simulink model "space_vector_current_control"  (Simulink 7.5)
settings: Solver=ode23tb  StartTime=0.0  StopTime=0.2  FixedStep=1e-5  MaxStep=1e-4  RelTol=1e-4  AbsTol=1e-6
libraries: simulink x40, powerlib x35
settings Model: Creator=ankush  LastModifiedBy=ankush

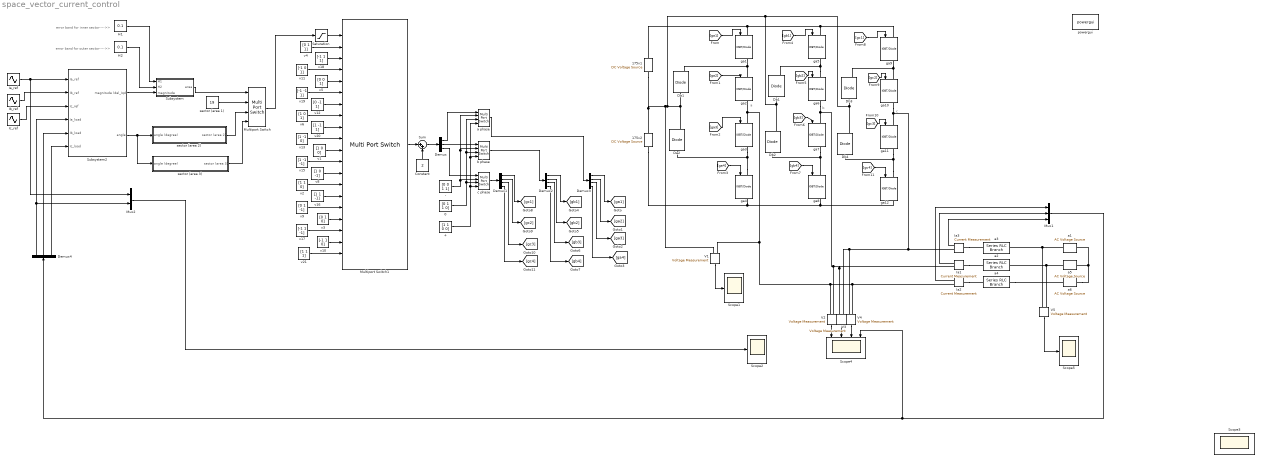
== system space_vector_current_control ==
  note: a
  note: b
  note: c
  note: error band for inner sector---->>
  note: error band for outer sector---->>
  + : Constant  Value=[1 1 0 0]  VectorParams1D=off  OutDataType=fixdt(1, 16)  OutScaling=2^0
  - : Constant  Value=[0 0 1 1]  OutDataType=fixdt(1, 16)  OutScaling=2^0
  0 : Constant  Value=[0 1 1 0]  OutDataType=fixdt(1, 16)  OutScaling=2^0
  175v1 : powerlib/Electrical Sources/DC Voltage Source  DialogController=POWERSYS.PowerSysDialog  SystemSampleTime=-1  Amplitude=300  Measurements=None
  175v2 : powerlib/Electrical Sources/DC Voltage Source  DialogController=POWERSYS.PowerSysDialog  SystemSampleTime=-1  Amplitude=300  Measurements=None
  Constant : Constant  Value=2  OutDataType=fixdt(1, 16)  OutScaling=2^0
  Da1 : powerlib/Power Electronics/Diode  DialogController=POWERSYS.PowerSysDialog  SystemSampleTime=-1  Ron=0.001  Lon=0  Vf=0.8  IC=0  UseSnubber=off  Rs=500  Cs=250e-9  Measurements=on
  Da2 : powerlib/Power Electronics/Diode  DialogController=POWERSYS.PowerSysDialog  SystemSampleTime=-1  Ron=0.001  Lon=0  Vf=0.8  IC=0  UseSnubber=off  Rs=500  Cs=250e-9  Measurements=on
  Db{1..4} (4 alike) : powerlib/Power Electronics/Diode  DialogController=POWERSYS.PowerSysDialog  SystemSampleTime=-1  Ron=0.001  Lon=0  Vf=0.8  IC=0  UseSnubber=off  Rs=500  Cs=250e-9  Measurements=on
  Demux : Demux  Outputs=3
  Demux1 : Demux
  Demux2 : Demux
  Demux3 : Demux
  Demux4 : Demux  Outputs=3
  H1 : Constant  Value=0.1  OutDataType=fixdt(1, 16)  OutScaling=2^0
  H2 : Constant  Value=0.1  OutDataType=fixdt(1, 16)  OutScaling=2^0
  Ia1 : powerlib/Measurements/Current Measurement  DialogController=POWERSYS.PowerSysDialog  SystemSampleTime=-1  PhasorSimulation=off  OutputType=Complex  PSBequivalent=0
  Ia2 : powerlib/Measurements/Current Measurement  DialogController=POWERSYS.PowerSysDialog  SystemSampleTime=-1  PhasorSimulation=off  OutputType=Complex  PSBequivalent=0
  Ia3 : powerlib/Measurements/Current Measurement  DialogController=POWERSYS.PowerSysDialog  SystemSampleTime=-1  PhasorSimulation=off  OutputType=Complex  PSBequivalent=0
  Ia_ref : Sin  Amplitude=5  Bias=0  Frequency=2*pi*50  Phase=0  Samples=10  SampleTime=0  Offset=0
  Ib_ref : Sin  Amplitude=5  Bias=0  Frequency=2*pi*50  Phase=-2*pi/3  Samples=10  SampleTime=0  Offset=0
  Ic_ref : Sin  Amplitude=5  Bias=0  Frequency=2*pi*50  Phase=2*pi/3  Samples=10  SampleTime=0  Offset=0
  Multiport Switch : MultiPortSwitch  zeroidx=off  OutDataType=fixdt(1, 16)  OutScaling=2^0
  Multiport Switch1 : MultiPortSwitch  Inputs=19  zeroidx=off  OutDataType=fixdt(1, 16)  OutScaling=2^0
  Mux1 : Mux  Inputs=3
  Mux2 : Mux  Inputs=2
  Saturation : Saturate  UpperLimit=19  LowerLimit=1  OutDataType=fixdt(1, 16)  OutScaling=2^0
  Scope1 : Scope
      settings: TimeRange=0.1  YMin=-200  YMax=175  SaveName=ScopeData3
  Scope2 : Scope
      settings: TimeRange=0.5  YMin=-5.5  YMax=5.5  SaveName=ScopeData2
  Scope3 : Scope  NumInputPorts=4
      settings: YMin=-5~-400~-350~-400  YMax=5~400~350~400
  Scope4 : Scope  NumInputPorts=4
      settings: YMin=-700~-700~-700~-7.5  YMax=700~700~700~7.5
  Scope5 : Scope
      settings: TimeRange=0.1  YMin=-600  YMax=600  SaveName=ScopeData6
  Subsystem : Subsystem
  Subsystem2 : Subsystem
  Sum : Sum  Inputs=|++  OutDataType=fixdt(1, 16)  OutScaling=2^0
  V{1..5} (5 alike) : powerlib/Measurements/Voltage Measurement  DialogController=POWERSYS.PowerSysDialog  SystemSampleTime=-1  PhasorSimulation=off  OutputType=Complex  PSBequivalent=0
  a phase : MultiPortSwitch  zeroidx=off  OutDataType=fixdt(1, 16)  OutScaling=2^0
  a1 : powerlib/Electrical Sources/AC Voltage Source  DialogController=POWERSYS.PowerSysDialog  SystemSampleTime=-1  Amplitude=240*sqrt(2)  Phase=120 + 88.178  Frequency=50  SampleTime=0  Measurements=None
  a2 : powerlib/Elements/Series RLC Branch  DialogController=POWERSYS.PowerSysDialog  PhysicalDomain=powersysdomain  SubClassName=unknown  LeftPortType=p1  RightPortType=p1  LConnTagsString=__new0  RConnTagsString=__new0  BranchType=RL  Resistance=0.03  Inductance=3e-3  SetiL0=off  InitialCurrent=0  Capacitance=2000e-6  Setx0=off  InitialVoltage=0  Measurements=None
  a3 : powerlib/Elements/Series RLC Branch  DialogController=POWERSYS.PowerSysDialog  PhysicalDomain=powersysdomain  SubClassName=unknown  LeftPortType=p1  RightPortType=p1  LConnTagsString=__new0  RConnTagsString=__new0  BranchType=RL  Resistance=0.03  Inductance=3e-3  SetiL0=off  InitialCurrent=0  Capacitance=2000e-6  Setx0=off  InitialVoltage=0  Measurements=None
  a4 : powerlib/Elements/Series RLC Branch  DialogController=POWERSYS.PowerSysDialog  PhysicalDomain=powersysdomain  SubClassName=unknown  LeftPortType=p1  RightPortType=p1  LConnTagsString=__new0  RConnTagsString=__new0  BranchType=RL  Resistance=0.03  Inductance=3e-3  SetiL0=off  InitialCurrent=0  Capacitance=2000e-6  Setx0=off  InitialVoltage=0  Measurements=None
  a5 : powerlib/Electrical Sources/AC Voltage Source  DialogController=POWERSYS.PowerSysDialog  SystemSampleTime=-1  Amplitude=240*sqrt(2)  Phase=-120 + 88.178  Frequency=50  SampleTime=0  Measurements=None
  a6 : powerlib/Electrical Sources/AC Voltage Source  DialogController=POWERSYS.PowerSysDialog  SystemSampleTime=-1  Amplitude=240*sqrt(2)  Phase=88.178  Frequency=50  SampleTime=0  Measurements=None
  b phase : MultiPortSwitch  zeroidx=off  OutDataType=fixdt(1, 16)  OutScaling=2^0
  c phase : MultiPortSwitch  zeroidx=off  OutDataType=fixdt(1, 16)  OutScaling=2^0
  ga{1..12} (12 alike) : powerlib/Power Electronics/IGBT//Diode  DialogController=POWERSYS.PowerSysDialog  SystemSampleTime=-1  Ron=1e-3  Rs=1e5  Cs=inf  Measurements=on
  powergui : powerlib/powergui  Priority=1  SystemSampleTime=-1  SimulationMode=Discrete  SampleTime=5e-6  frequency=60  SPID=off  DisableSnubberDevices=off  DisableRonSwitches=off  DisableVfSwitches=off  SwTol=0  Interpol=off  frequencyindice=0  echomessages=off  HookPort=off  DisplayEquations=off  FunctionMessages=off  EnableUseOfTLC=off  x0status=blocks  RestoreLinks=warning  ResistiveCurrentMeasurement=off  Ylog=off  Xlog=on  ShowGrid=off  save=off  variable=ZData  ZoomFFT=off  StartTime=0.0  cycles=1  DisplayStyle=1  FreqAxis=off  MaxFrequency=1000  frequencyindicesteady=1  display=off  methode=off
  sector (area 1) : Constant  Value=19  OutDataType=fixdt(1, 16)  OutScaling=2^0
  sector (area 2) : Subsystem
  sector (area 3) : Subsystem
  v1 : Constant  Value=[1 0 0]  VectorParams1D=off  OutDataType=fixdt(1, 16)  OutScaling=2^0
  v10 : Constant  Value=[-1 1 0]  VectorParams1D=off  OutDataType=fixdt(1, 16)  OutScaling=2^0
  v11 : Constant  Value=[-1 0 1]  VectorParams1D=off  OutDataType=fixdt(1, 16)  OutScaling=2^0
  v12 : Constant  Value=[0 -1 1]  VectorParams1D=off  OutDataType=fixdt(1, 16)  OutScaling=2^0
  v13 : Constant  Value=[1 -1 0]  VectorParams1D=off  OutDataType=fixdt(1, 16)  OutScaling=2^0
  v15 : Constant  Value=[1 -1 -1]  VectorParams1D=off  OutDataType=fixdt(1, 16)  OutScaling=2^0
  v16 : Constant  Value=[1 1 -1]  VectorParams1D=off  OutDataType=fixdt(1, 16)  OutScaling=2^0
  v17 : Constant  Value=[-1 1 -1]  VectorParams1D=off  OutDataType=fixdt(1, 16)  OutScaling=2^0
  v18 : Constant  Value=[-1 1 1]  VectorParams1D=off  OutDataType=fixdt(1, 16)  OutScaling=2^0
  v19 : Constant  Value=[-1 -1 1]  VectorParams1D=off  OutDataType=fixdt(1, 16)  OutScaling=2^0
  v2 : Constant  Value=[1 1 0]  VectorParams1D=off  OutDataType=fixdt(1, 16)  OutScaling=2^0
  v20 : Constant  Value=[1 -1 1]  VectorParams1D=off  OutDataType=fixdt(1, 16)  OutScaling=2^0
  v21 : Constant  Value=[1 1 1]  VectorParams1D=off  OutDataType=fixdt(1, 16)  OutScaling=2^0
  v3 : Constant  Value=[0 1 0]  VectorParams1D=off  OutDataType=fixdt(1, 16)  OutScaling=2^0
  v4 : Constant  Value=[0 1 1]  VectorParams1D=off  OutDataType=fixdt(1, 16)  OutScaling=2^0
  v5 : Constant  Value=[0 0 1]  VectorParams1D=off  OutDataType=fixdt(1, 16)  OutScaling=2^0
  v6 : Constant  Value=[1 0 1]  VectorParams1D=off  OutDataType=fixdt(1, 16)  OutScaling=2^0
  v8 : Constant  Value=[1 0 -1]  VectorParams1D=off  OutDataType=fixdt(1, 16)  OutScaling=2^0
  v9 : Constant  Value=[0 1 -1]  VectorParams1D=off  OutDataType=fixdt(1, 16)  OutScaling=2^0
  wires:
  sector (area 1)/1 -> Multiport Switch/2
  sector (area 2)/1(sector (area 2)) -> Multiport Switch/3
  sector (area 3)/1(sector (area 3)) -> Multiport Switch/4
  Multiport Switch/1 -> Saturation/1
  Ia_ref/1 -> Mux2/1, Subsystem2/1(Ia_ref)
  Ib_ref/1 -> Subsystem2/2(Ib_ref)
  Ic_ref/1 -> Subsystem2/3(Ic_ref)
  Sum/1 -> Demux/1
  Demux/2 -> b phase/1
  +/1 -> c phase/4, b phase/4, a phase/4
  0/1 -> c phase/3, a phase/3, b phase/3
  -/1 -> a phase/2, b phase/2, c phase/2
  c phase/1 -> Demux1/1
  Demux1/1 -> [gc1]
  Demux1/4 -> [gc4]
  b phase/1 -> Demux2/1
  Demux1/2 -> [gc2]
  Demux1/3 -> [gc3]
  Demux2/4 -> [gb4]
  Demux2/3 -> [gb3]
  Demux2/2 -> [gb2]
  Demux2/1 -> [gb1]
  a phase/1 -> Demux3/1
  Demux3/4 -> [ga4]
  Demux3/3 -> [ga3]
  Demux3/2 -> [ga2]
  Demux3/1 -> [ga1]
  Constant/1 -> Sum/2
  Multiport Switch1/1 -> Sum/1
  [ga1] -> ga1/1
  [ga2] -> ga2/1
  [ga3] -> ga3/1
  [ga4] -> ga4/1
  [gb1] -> ga5/1
  [gb2] -> ga6/1
  [gb3] -> ga7/1
  [gb4] -> ga8/1
  [gc1] -> ga9/1
  [gc2] -> ga10/1
  [gc3] -> ga11/1
  [gc4] -> ga12/1
  V4/1 -> Scope4/3
  V3/1 -> Scope4/2
  V2/1 -> Scope4/1
  Subsystem2/1(magnitude (del_Iqd)) -> Subsystem/3(magnitude)
  v10/1 -> Multiport Switch1/19
  v17/1 -> Multiport Switch1/18
  v9/1 -> Multiport Switch1/16
  v16/1 -> Multiport Switch1/15
  v8/1 -> Multiport Switch1/13
  v15/1 -> Multiport Switch1/12
  v13/1 -> Multiport Switch1/10
  v20/1 -> Multiport Switch1/9
  v12/1 -> Multiport Switch1/7
  v19/1 -> Multiport Switch1/6
  v11/1 -> Multiport Switch1/4
  v18/1 -> Multiport Switch1/3
  v3/1 -> Multiport Switch1/17
  v2/1 -> Multiport Switch1/14
  v1/1 -> Multiport Switch1/11
  v6/1 -> Multiport Switch1/8
  v5/1 -> Multiport Switch1/5
  v4/1 -> Multiport Switch1/2
  Mux2/1 -> Scope2/1
  Demux/3 -> c phase/1
  Demux/1 -> a phase/1
  v21/1 -> Multiport Switch1/20
  Saturation/1 -> Multiport Switch1/1
  Demux4/1 -> Subsystem2/4(Ia_load), Mux2/2
  Demux4/2 -> Subsystem2/5(Ib_load)
  Demux4/3 -> Subsystem2/6(Ic_load)
  H1/1 -> Subsystem/1(H1)
  H2/1 -> Subsystem/2(H2)
  Subsystem2/2(angle) -> sector (area 2)/1(angle (degree)), sector (area 3)/1(angle (degree))
  Subsystem/1(area) -> Multiport Switch/1
  V1/1 -> Scope1/1
  Mux1/1 -> Demux4/1, Scope4/4
  Ia2/1 -> Mux1/1
  Ia1/1 -> Mux1/2
  Ia3/1 -> Mux1/3
  V5/1 -> Scope5/1
  connections:
  ga1/RConn1 -- Da1/RConn1 -- ga2/LConn1
  ga4/LConn1 -- Da2/LConn1 -- ga3/RConn1
  175v1/RConn1 -- ga1/LConn1 -- ga5/LConn1 -- ga9/LConn1
  ga12/RConn1 -- ga4/RConn1 -- 175v2/LConn1 -- ga8/RConn1
  ga6/LConn1 -- Db1/RConn1 -- ga5/RConn1
  Db2/LConn1 -- ga8/LConn1 -- ga7/RConn1
  Db3/RConn1 -- ga10/LConn1 -- ga9/RConn1
  ga12/LConn1 -- Db4/LConn1 -- ga11/RConn1
  V3/LConn2 -- V4/LConn1 -- ga10/RConn1 -- ga11/LConn1 -- Ia3/RConn1
  V4/LConn2 -- ga3/LConn1 -- ga2/RConn1 -- V1/LConn2 -- V2/LConn1 -- Ia2/RConn1
  V3/LConn1 -- ga7/LConn1 -- ga6/RConn1 -- V2/LConn2 -- Ia1/RConn1
  175v1/LConn1 -- 175v2/RConn1 -- Db3/LConn1 -- Db4/RConn1 -- Db2/RConn1 -- Db1/LConn1 -- Da2/RConn1 -- Da1/LConn1 -- V1/LConn1
  a6/LConn1 -- a1/LConn1 -- a5/LConn1
  Ia3/LConn1 -- a3/RConn1
  Ia2/LConn1 -- a4/RConn1
  Ia1/LConn1 -- a2/RConn1
  a4/LConn1 -- a6/RConn1
  a5/RConn1 -- a2/LConn1 -- V5/LConn2
  a1/RConn1 -- a3/LConn1 -- V5/LConn1

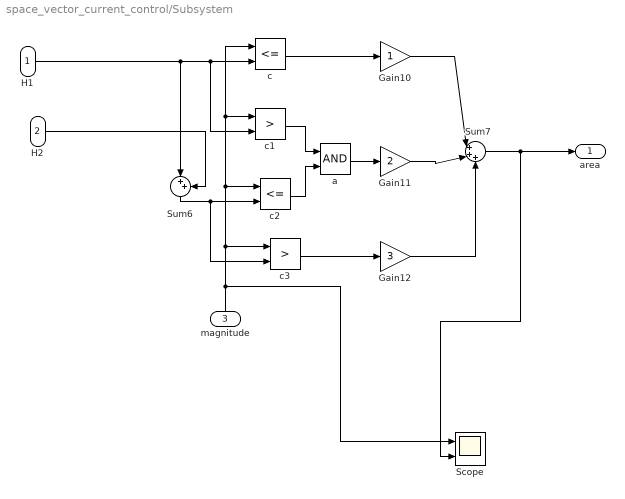
== system space_vector_current_control/Subsystem ==
  H1 : Inport
  H2 : Inport  Port=2
  magnitude : Inport  Port=3
  Gain10 : Gain  ParameterDataType=fixdt(1, 16)  ParameterScaling=2^0  OutDataType=fixdt(1, 16)  OutScaling=2^0
  Gain11 : Gain  Gain=2  ParameterDataType=fixdt(1, 16)  ParameterScaling=2^0  OutDataType=fixdt(1, 16)  OutScaling=2^0
  Gain12 : Gain  Gain=3  ParameterDataType=fixdt(1, 16)  ParameterScaling=2^0  OutDataType=fixdt(1, 16)  OutScaling=2^0
  Scope : Scope  NumInputPorts=2
      settings: YMin=-1.73472e-017~1  YMax=0.23~3  SaveName=ScopeData4
  Sum6 : Sum  Inputs=|++  OutDataType=fixdt(1, 16)  OutScaling=2^0
  Sum7 : Sum  Inputs=|+++  OutDataType=fixdt(1, 16)  OutScaling=2^0
  a : Logic  AllPortsSameDT=off  OutDataTypeMode=boolean  LogicDataType=fixdt(0, 8)  OutDataTypeStr=boolean
  c : RelationalOperator  Operator=<=  LogicOutDataTypeMode=boolean  LogicDataType=fixdt(0, 8)  OutDataTypeStr=boolean
  c1 : RelationalOperator  Operator=>  LogicOutDataTypeMode=boolean  LogicDataType=fixdt(0, 8)  OutDataTypeStr=boolean
  c2 : RelationalOperator  Operator=<=  LogicOutDataTypeMode=boolean  LogicDataType=fixdt(0, 8)  OutDataTypeStr=boolean
  c3 : RelationalOperator  Operator=>  LogicOutDataTypeMode=boolean  LogicDataType=fixdt(0, 8)  OutDataTypeStr=boolean
  area : Outport
  wires:
  H1/1 -> Sum6/1, c/2, c1/2
  c/1 -> Gain10/1
  H2/1 -> Sum6/2
  Sum6/1 -> c2/2, c3/2
  c1/1 -> a/1
  c2/1 -> a/2
  a/1 -> Gain11/1
  c3/1 -> Gain12/1
  Gain10/1 -> Sum7/1
  Gain11/1 -> Sum7/2
  Gain12/1 -> Sum7/3
  magnitude/1 -> c/1, c1/1, c2/1, c3/1, Scope/1
  Sum7/1 -> area/1, Scope/2

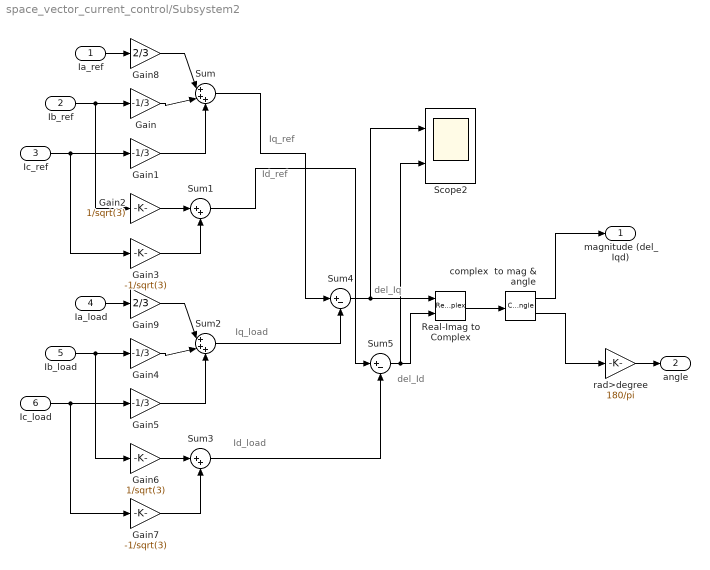
== system space_vector_current_control/Subsystem2 ==
  note: Iq_ref
  note: Id_ref
  note: Iq_load
  note: Id_load
  note: del_Iq
  note: del_Id
  Ia_ref : Inport
  Ib_ref : Inport  Port=2
  Ic_ref : Inport  Port=3
  Ia_load : Inport  Port=4
  Ib_load : Inport  Port=5
  Ic_load : Inport  Port=6
  Gain{,1,4..5} (4 alike) : Gain  Gain=-1/3  ParameterDataType=fixdt(1, 16)  ParameterScaling=2^0  OutDataType=fixdt(1, 16)  OutScaling=2^0
  Gain2 : Gain  Gain=1/sqrt(3)  ParameterDataType=fixdt(1, 16)  ParameterScaling=2^0  OutDataType=fixdt(1, 16)  OutScaling=2^0
  Gain3 : Gain  Gain=-1/sqrt(3)  ParameterDataType=fixdt(1, 16)  ParameterScaling=2^0  OutDataType=fixdt(1, 16)  OutScaling=2^0
  Gain6 : Gain  Gain=1/sqrt(3)  ParameterDataType=fixdt(1, 16)  ParameterScaling=2^0  OutDataType=fixdt(1, 16)  OutScaling=2^0
  Gain7 : Gain  Gain=-1/sqrt(3)  ParameterDataType=fixdt(1, 16)  ParameterScaling=2^0  OutDataType=fixdt(1, 16)  OutScaling=2^0
  Gain8 : Gain  Gain=2/3  ParameterDataType=fixdt(1, 16)  ParameterScaling=2^0  OutDataType=fixdt(1, 16)  OutScaling=2^0
  Gain9 : Gain  Gain=2/3  ParameterDataType=fixdt(1, 16)  ParameterScaling=2^0  OutDataType=fixdt(1, 16)  OutScaling=2^0
  Real-Imag to Complex : RealImagToComplex
  Scope2 : Scope  NumInputPorts=2
      settings: YMin=0.5~-12  YMax=9~-1.5  SaveName=ScopeData5
  Sum : Sum  Inputs=|+++  OutDataType=fixdt(1, 16)  OutScaling=2^0
  Sum1 : Sum  Inputs=|++  OutDataType=fixdt(1, 16)  OutScaling=2^0
  Sum2 : Sum  Inputs=|+++  OutDataType=fixdt(1, 16)  OutScaling=2^0
  Sum3 : Sum  Inputs=|++  OutDataType=fixdt(1, 16)  OutScaling=2^0
  Sum4 : Sum  Inputs=|+-  OutDataType=fixdt(1, 16)  OutScaling=2^0
  Sum5 : Sum  Inputs=|+-  OutDataType=fixdt(1, 16)  OutScaling=2^0
  complex  to mag & angle : ComplexToMagnitudeAngle
  rad>degree : Gain  Gain=180/pi  ParameterDataType=fixdt(1, 16)  ParameterScaling=2^0  OutDataType=fixdt(1, 16)  OutScaling=2^0
  magnitude (del_Iqd) : Outport
  angle : Outport  Port=2
  wires:
  Gain/1 -> Sum/2
  Gain1/1 -> Sum/3
  Ib_ref/1 -> Gain2/1, Gain/1
  Ic_ref/1 -> Gain3/1, Gain1/1
  Gain2/1 -> Sum1/1
  Gain3/1 -> Sum1/2
  Sum/1 -> Sum4/1
  Sum1/1 -> Sum5/1
  Gain4/1 -> Sum2/2
  Gain5/1 -> Sum2/3
  Ib_load/1 -> Gain4/1, Gain6/1
  Ic_load/1 -> Gain5/1, Gain7/1
  Gain6/1 -> Sum3/1
  Gain7/1 -> Sum3/2
  Sum2/1 -> Sum4/2
  Sum3/1 -> Sum5/2
  Real-Imag to Complex/1 -> complex  to mag & angle/1
  Sum4/1 -> Real-Imag to Complex/1, Scope2/1
  Sum5/1 -> Real-Imag to Complex/2, Scope2/2
  Gain8/1 -> Sum/1
  Gain9/1 -> Sum2/1
  Ia_ref/1 -> Gain8/1
  Ia_load/1 -> Gain9/1
  rad>degree/1 -> angle/1
  complex  to mag & angle/2 -> rad>degree/1
  complex  to mag & angle/1 -> magnitude (del_Iqd)/1

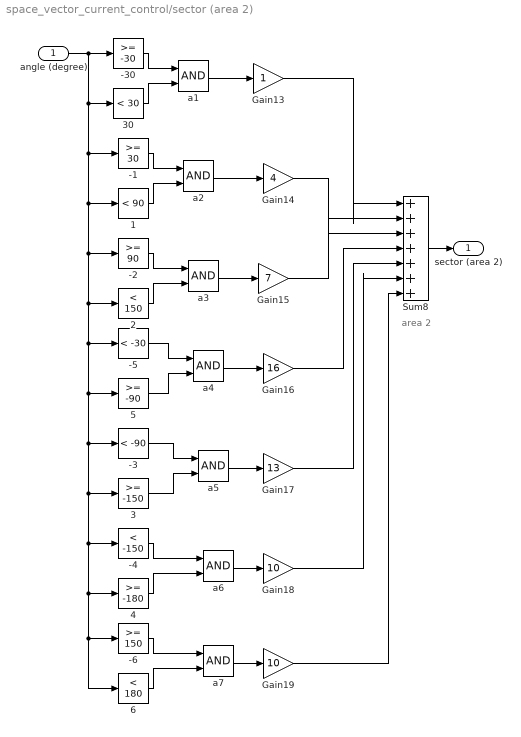
== system space_vector_current_control/sector (area 2) ==
  note: area 2
  angle (degree) : Inport
  -1 : simulink/Logic and Bit Operations/Compare To Constant  SystemSampleTime=-1  relop=>=  const=30  LogicOutDataTypeMode=uint8
  -2 : simulink/Logic and Bit Operations/Compare To Constant  SystemSampleTime=-1  relop=>=  const=90  LogicOutDataTypeMode=uint8
  -3 : simulink/Logic and Bit Operations/Compare To Constant  SystemSampleTime=-1  relop=<  const=-90  LogicOutDataTypeMode=uint8
  -30 : simulink/Logic and Bit Operations/Compare To Constant  SystemSampleTime=-1  relop=>=  const=-30  LogicOutDataTypeMode=uint8
  -4 : simulink/Logic and Bit Operations/Compare To Constant  SystemSampleTime=-1  relop=<  const=-150  LogicOutDataTypeMode=uint8
  -5 : simulink/Logic and Bit Operations/Compare To Constant  SystemSampleTime=-1  relop=<  const=-30  LogicOutDataTypeMode=uint8
  -6 : simulink/Logic and Bit Operations/Compare To Constant  SystemSampleTime=-1  relop=>=  const=150  LogicOutDataTypeMode=uint8
  1 : simulink/Logic and Bit Operations/Compare To Constant  SystemSampleTime=-1  relop=<  const=90  LogicOutDataTypeMode=uint8
  2 : simulink/Logic and Bit Operations/Compare To Constant  SystemSampleTime=-1  relop=<  const=150  LogicOutDataTypeMode=uint8
  3 : simulink/Logic and Bit Operations/Compare To Constant  SystemSampleTime=-1  relop=>=  const=-150  LogicOutDataTypeMode=uint8
  30 : simulink/Logic and Bit Operations/Compare To Constant  SystemSampleTime=-1  relop=<  const=30  LogicOutDataTypeMode=uint8
  4 : simulink/Logic and Bit Operations/Compare To Constant  SystemSampleTime=-1  relop=>=  const=-180  LogicOutDataTypeMode=uint8
  5 : simulink/Logic and Bit Operations/Compare To Constant  SystemSampleTime=-1  relop=>=  const=-90  LogicOutDataTypeMode=uint8
  6 : simulink/Logic and Bit Operations/Compare To Constant  SystemSampleTime=-1  relop=<  const=180  LogicOutDataTypeMode=uint8
  Gain13 : Gain  ParameterDataType=fixdt(1, 16)  ParameterScaling=2^0  OutDataType=fixdt(1, 16)  OutScaling=2^0
  Gain14 : Gain  Gain=4  ParameterDataType=fixdt(1, 16)  ParameterScaling=2^0  OutDataType=fixdt(1, 16)  OutScaling=2^0
  Gain15 : Gain  Gain=7  ParameterDataType=fixdt(1, 16)  ParameterScaling=2^0  OutDataType=fixdt(1, 16)  OutScaling=2^0
  Gain16 : Gain  Gain=16  ParameterDataType=fixdt(1, 16)  ParameterScaling=2^0  OutDataType=fixdt(1, 16)  OutScaling=2^0
  Gain17 : Gain  Gain=13  ParameterDataType=fixdt(1, 16)  ParameterScaling=2^0  OutDataType=fixdt(1, 16)  OutScaling=2^0
  Gain18 : Gain  Gain=10  ParameterDataType=fixdt(1, 16)  ParameterScaling=2^0  OutDataType=fixdt(1, 16)  OutScaling=2^0
  Gain19 : Gain  Gain=10  ParameterDataType=fixdt(1, 16)  ParameterScaling=2^0  OutDataType=fixdt(1, 16)  OutScaling=2^0
  Sum8 : Sum  Inputs=|+++++++  OutDataType=fixdt(1, 16)  OutScaling=2^0
  a{1..7} (7 alike) : Logic  AllPortsSameDT=off  OutDataTypeMode=boolean  LogicDataType=fixdt(0, 8)  OutDataTypeStr=boolean
  sector (area 2) : Outport
  wires:
  -30/1 -> a1/1
  30/1 -> a1/2
  -1/1 -> a2/1
  1/1 -> a2/2
  -2/1 -> a3/1
  2/1 -> a3/2
  -5/1 -> a4/1
  5/1 -> a4/2
  -3/1 -> a5/1
  3/1 -> a5/2
  -4/1 -> a6/1
  4/1 -> a6/2
  a1/1 -> Gain13/1
  a2/1 -> Gain14/1
  a3/1 -> Gain15/1
  a4/1 -> Gain16/1
  a5/1 -> Gain17/1
  a6/1 -> Gain18/1
  Gain13/1 -> Sum8/1
  Gain14/1 -> Sum8/2
  Gain15/1 -> Sum8/3
  Gain16/1 -> Sum8/4
  Gain17/1 -> Sum8/5
  Gain18/1 -> Sum8/6
  -6/1 -> a7/1
  6/1 -> a7/2
  a7/1 -> Gain19/1
  Gain19/1 -> Sum8/7
  angle (degree)/1 -> -30/1, 30/1, -1/1, 1/1, -2/1, 2/1, -5/1, 5/1, -3/1, 3/1, -4/1, 4/1, -6/1, 6/1
  Sum8/1 -> sector (area 2)/1

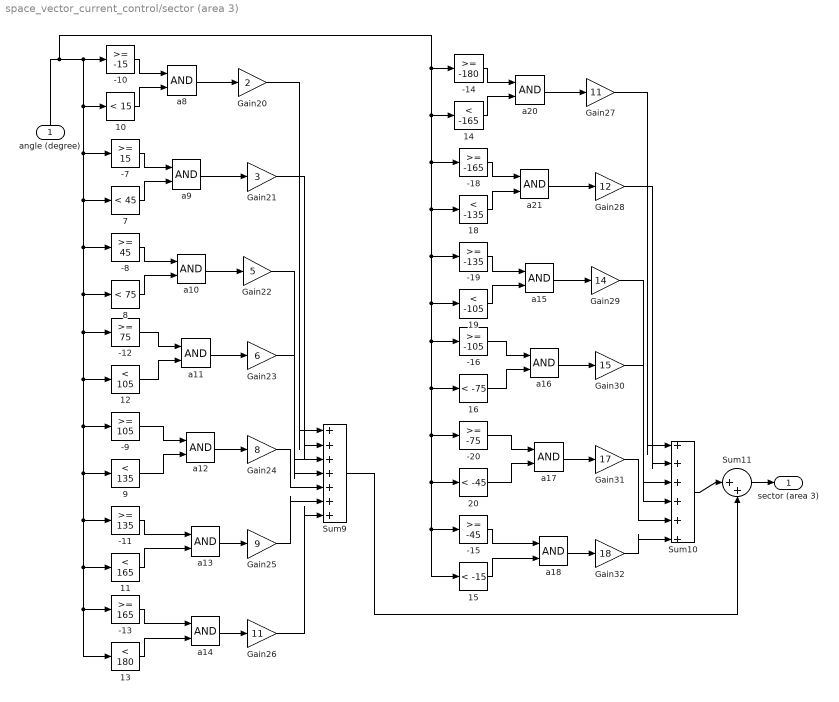
== system space_vector_current_control/sector (area 3) ==
  angle (degree) : Inport
  -10 : simulink/Logic and Bit Operations/Compare To Constant  SystemSampleTime=-1  relop=>=  const=-15  LogicOutDataTypeMode=uint8
  -11 : simulink/Logic and Bit Operations/Compare To Constant  SystemSampleTime=-1  relop=>=  const=135  LogicOutDataTypeMode=uint8
  -12 : simulink/Logic and Bit Operations/Compare To Constant  SystemSampleTime=-1  relop=>=  const=75  LogicOutDataTypeMode=uint8
  -13 : simulink/Logic and Bit Operations/Compare To Constant  SystemSampleTime=-1  relop=>=  const=165  LogicOutDataTypeMode=uint8
  -14 : simulink/Logic and Bit Operations/Compare To Constant  SystemSampleTime=-1  relop=>=  const=-180  LogicOutDataTypeMode=uint8
  -15 : simulink/Logic and Bit Operations/Compare To Constant  SystemSampleTime=-1  relop=>=  const=-45  LogicOutDataTypeMode=uint8
  -16 : simulink/Logic and Bit Operations/Compare To Constant  SystemSampleTime=-1  relop=>=  const=-105  LogicOutDataTypeMode=uint8
  -18 : simulink/Logic and Bit Operations/Compare To Constant  SystemSampleTime=-1  relop=>=  const=-165  LogicOutDataTypeMode=uint8
  -19 : simulink/Logic and Bit Operations/Compare To Constant  SystemSampleTime=-1  relop=>=  const=-135  LogicOutDataTypeMode=uint8
  -20 : simulink/Logic and Bit Operations/Compare To Constant  SystemSampleTime=-1  relop=>=  const=-75  LogicOutDataTypeMode=uint8
  -7 : simulink/Logic and Bit Operations/Compare To Constant  SystemSampleTime=-1  relop=>=  const=15  LogicOutDataTypeMode=uint8
  -8 : simulink/Logic and Bit Operations/Compare To Constant  SystemSampleTime=-1  relop=>=  const=45  LogicOutDataTypeMode=uint8
  -9 : simulink/Logic and Bit Operations/Compare To Constant  SystemSampleTime=-1  relop=>=  const=105  LogicOutDataTypeMode=uint8
  10 : simulink/Logic and Bit Operations/Compare To Constant  SystemSampleTime=-1  relop=<  const=15  LogicOutDataTypeMode=uint8
  11 : simulink/Logic and Bit Operations/Compare To Constant  SystemSampleTime=-1  relop=<  const=165  LogicOutDataTypeMode=uint8
  12 : simulink/Logic and Bit Operations/Compare To Constant  SystemSampleTime=-1  relop=<  const=105  LogicOutDataTypeMode=uint8
  13 : simulink/Logic and Bit Operations/Compare To Constant  SystemSampleTime=-1  relop=<  const=180  LogicOutDataTypeMode=uint8
  14 : simulink/Logic and Bit Operations/Compare To Constant  SystemSampleTime=-1  relop=<  const=-165  LogicOutDataTypeMode=uint8
  15 : simulink/Logic and Bit Operations/Compare To Constant  SystemSampleTime=-1  relop=<  const=-15  LogicOutDataTypeMode=uint8
  16 : simulink/Logic and Bit Operations/Compare To Constant  SystemSampleTime=-1  relop=<  const=-75  LogicOutDataTypeMode=uint8
  18 : simulink/Logic and Bit Operations/Compare To Constant  SystemSampleTime=-1  relop=<  const=-135  LogicOutDataTypeMode=uint8
  19 : simulink/Logic and Bit Operations/Compare To Constant  SystemSampleTime=-1  relop=<  const=-105  LogicOutDataTypeMode=uint8
  20 : simulink/Logic and Bit Operations/Compare To Constant  SystemSampleTime=-1  relop=<  const=-45  LogicOutDataTypeMode=uint8
  7 : simulink/Logic and Bit Operations/Compare To Constant  SystemSampleTime=-1  relop=<  const=45  LogicOutDataTypeMode=uint8
  8 : simulink/Logic and Bit Operations/Compare To Constant  SystemSampleTime=-1  relop=<  const=75  LogicOutDataTypeMode=uint8
  9 : simulink/Logic and Bit Operations/Compare To Constant  SystemSampleTime=-1  relop=<  const=135  LogicOutDataTypeMode=uint8
  Gain20 : Gain  Gain=2  ParameterDataType=fixdt(1, 16)  ParameterScaling=2^0  OutDataType=fixdt(1, 16)  OutScaling=2^0
  Gain21 : Gain  Gain=3  ParameterDataType=fixdt(1, 16)  ParameterScaling=2^0  OutDataType=fixdt(1, 16)  OutScaling=2^0
  Gain22 : Gain  Gain=5  ParameterDataType=fixdt(1, 16)  ParameterScaling=2^0  OutDataType=fixdt(1, 16)  OutScaling=2^0
  Gain23 : Gain  Gain=6  ParameterDataType=fixdt(1, 16)  ParameterScaling=2^0  OutDataType=fixdt(1, 16)  OutScaling=2^0
  Gain24 : Gain  Gain=8  ParameterDataType=fixdt(1, 16)  ParameterScaling=2^0  OutDataType=fixdt(1, 16)  OutScaling=2^0
  Gain25 : Gain  Gain=9  ParameterDataType=fixdt(1, 16)  ParameterScaling=2^0  OutDataType=fixdt(1, 16)  OutScaling=2^0
  Gain26 : Gain  Gain=11  ParameterDataType=fixdt(1, 16)  ParameterScaling=2^0  OutDataType=fixdt(1, 16)  OutScaling=2^0
  Gain27 : Gain  Gain=11  ParameterDataType=fixdt(1, 16)  ParameterScaling=2^0  OutDataType=fixdt(1, 16)  OutScaling=2^0
  Gain28 : Gain  Gain=12  ParameterDataType=fixdt(1, 16)  ParameterScaling=2^0  OutDataType=fixdt(1, 16)  OutScaling=2^0
  Gain29 : Gain  Gain=14  ParameterDataType=fixdt(1, 16)  ParameterScaling=2^0  OutDataType=fixdt(1, 16)  OutScaling=2^0
  Gain30 : Gain  Gain=15  ParameterDataType=fixdt(1, 16)  ParameterScaling=2^0  OutDataType=fixdt(1, 16)  OutScaling=2^0
  Gain31 : Gain  Gain=17  ParameterDataType=fixdt(1, 16)  ParameterScaling=2^0  OutDataType=fixdt(1, 16)  OutScaling=2^0
  Gain32 : Gain  Gain=18  ParameterDataType=fixdt(1, 16)  ParameterScaling=2^0  OutDataType=fixdt(1, 16)  OutScaling=2^0
  Sum10 : Sum  Inputs=|++++++  OutDataType=fixdt(1, 16)  OutScaling=2^0
  Sum11 : Sum  Inputs=|++  OutDataType=fixdt(1, 16)  OutScaling=2^0
  Sum9 : Sum  Inputs=|+++++++  OutDataType=fixdt(1, 16)  OutScaling=2^0
  a{8..18,20..21} (13 alike) : Logic  AllPortsSameDT=off  OutDataTypeMode=boolean  LogicDataType=fixdt(0, 8)  OutDataTypeStr=boolean
  sector (area 3) : Outport
  wires:
  -10/1 -> a8/1
  10/1 -> a8/2
  -7/1 -> a9/1
  7/1 -> a9/2
  -8/1 -> a10/1
  8/1 -> a10/2
  -12/1 -> a11/1
  12/1 -> a11/2
  -9/1 -> a12/1
  9/1 -> a12/2
  -11/1 -> a13/1
  11/1 -> a13/2
  a8/1 -> Gain20/1
  a9/1 -> Gain21/1
  a10/1 -> Gain22/1
  a11/1 -> Gain23/1
  a12/1 -> Gain24/1
  a13/1 -> Gain25/1
  -13/1 -> a14/1
  13/1 -> a14/2
  a14/1 -> Gain26/1
  Gain20/1 -> Sum9/1
  Gain21/1 -> Sum9/2
  Gain22/1 -> Sum9/3
  Gain23/1 -> Sum9/4
  Gain24/1 -> Sum9/5
  Gain25/1 -> Sum9/6
  Gain26/1 -> Sum9/7
  -14/1 -> a20/1
  14/1 -> a20/2
  -18/1 -> a21/1
  18/1 -> a21/2
  -19/1 -> a15/1
  19/1 -> a15/2
  -16/1 -> a16/1
  16/1 -> a16/2
  -20/1 -> a17/1
  20/1 -> a17/2
  -15/1 -> a18/1
  15/1 -> a18/2
  a20/1 -> Gain27/1
  a21/1 -> Gain28/1
  a15/1 -> Gain29/1
  a16/1 -> Gain30/1
  a17/1 -> Gain31/1
  a18/1 -> Gain32/1
  Gain27/1 -> Sum10/1
  Gain28/1 -> Sum10/2
  Gain29/1 -> Sum10/3
  Gain30/1 -> Sum10/4
  Gain31/1 -> Sum10/5
  Gain32/1 -> Sum10/6
  Sum10/1 -> Sum11/1
  Sum9/1 -> Sum11/2
  angle (degree)/1 -> -10/1, 10/1, -7/1, 7/1, -8/1, 8/1, -12/1, 12/1, -9/1, 9/1, -11/1, 11/1, -13/1, 13/1, -15/1, 15/1, 20/1, -20/1, 16/1, -16/1, 19/1, -19/1, 18/1, -18/1, 14/1, -14/1
  Sum11/1 -> sector (area 3)/1
